simulink model "gtm_design"  (R2020b)
settings: Solver=ode3  StartTime=0.0  StopTime=20  FixedStep=Timestep  MaxStep=0.1  MinStep=0.005  RelTol=1e-5
StopFcn:
  | MWSout=grabmws(bdroot);
  | MWSout.lastrun=datestr(now);
values from neighbouring files (symbols this model uses):
  AILL = simout.surf.AILL.Data    [plot_result.m]
  AILR = simout.surf.AILR.Data    [plot_result.m]
  ELLIB = simout.surf.ELLIB.Data    [plot_result.m]
  ELLOB = simout.surf.ELLOB.Data    [plot_result.m]
  ELRIB = simout.surf.ELRIB.Data    [plot_result.m]
  ELROB = simout.surf.ELROB.Data    [plot_result.m]
  RUDL = simout.surf.RUDL.Data    [plot_result.m]
  RUDU = simout.surf.RUDU.Data    [plot_result.m]
  THROTL = simout.surf.THROTL.Data    [plot_result.m]
  THROTR = simout.surf.THROTR.Data    [plot_result.m]
undefined symbols (not defined in the file or in its folder): Aero, aftfuel, aftfuel_pos, AILLC, AILRC, alpha_deg, altitude_ft, Ax_g, Ay_g, Az_g, b, beta_deg, bias, BRAKEC, Cbar, cg_pos0, cg_shift_gear, DamageCase, DamageModels, DamageOnsetTime, ELLIBC, ELLOBC, ELRIBC, ELROBC, engl_ang, engl_pos, engr_ang, engr_pos, FLAPLIB, FLAPLIC, FLAPLOB, FLAPLOC, FLAPRIB, FLAPRIC, FLAPROB, FLAPROC, FuelUsed_Init, fwdfuel, fwdfuel_pos, GEAR, GEARC, Inertia0, Inertia_shift_gear, Ixx_model, Iyy_model, Izz_model, KTAS, LandingGear, LengON, LinearizeModeOn, NAV_altitude_m, NAV_latitude_deg, NAV_longitude_deg, NAV_Ve_mps, NAV_Vn_mps, NAV_Vu_mps, Newton, p_deg, phi_deg, POS_hi ... (+40)
libraries: simulink_need_slupdate x40, simulink x4, simulink_extras x3, UserContent_lib x1
(part 1 of 6)
settings Model: ExtModeAutoUpdateStatusClock=off  OrderedModelArguments=off  Creator=cox  LastModifiedBy=Jihoon Lee
settings DataIOCC: LimitDataPoints=on  MaxDataPoints=50000  SaveFormat=Structure  SaveOutput=off  DSMLogging=off  ReturnWorkspaceOutputs=off
settings OptimizationCC: BooleanDataType=off  ExpressionDepthLimit=2147483647  InitFltsAndDblsToZero=on  LifeSpan=inf
settings DebuggingCC: AlgebraicLoopMsg=error  SaveWithParameterizedLinksMsg=none  MergeDetectMultiDrivingBlocksExec=none  SignalResolutionControl=TryResolveAllWithWarning  InheritedTsInSrcMsg=none  MultiTaskDSMMsg=warning  MultiTaskCondExecSysMsg=none  StateNameClashWarn=warning  InitInArrayFormatMsg=none  SFUnexpectedBacktrackingDiag=warning  SFNoUnconditionalDefaultTransitionDiag=warning  SFExecutionAtInitializationDiag=none  ArithmeticOperatorsInVariantConditions=warning
settings HardwareCC: ProdBitPerPointer=32  ProdBitPerSizeT=32  ProdBitPerPtrDiffT=32  ProdLargestAtomicFloat=None  ProdIntDivRoundTo=Undefined  ProdEndianess=Unspecified  ProdWordSize=32  ProdHWDeviceType=32-bit Generic  TargetHWDeviceType=32-bit Generic
settings ModelReferenceCC: PropagateSignalLabelsOutOfModel=off
settings SFSimCC: SimUseLocalCustomCode=off  SimParseCustomCode=off  CustomCodeUndefinedFunction=UseInterfaceOnly
settings RTWCC: RTWUseLocalCustomCode=off
settings CodeAppCC: StateflowObjectComments=on
settings GRTTargetCC: TargetFcnLib=ansi_tfl_tmw.mat  TargetLangStandard=C89/C90 (ANSI)  CombineOutputUpdateFcns=off  GRTInterface=on
settings ConfigComp: CovMetricSettings=dw  CovSaveCumulativeToWorkspaceVar=on  CovSaveSingleToWorkspaceVar=on  CovExternalEMLEnable=off

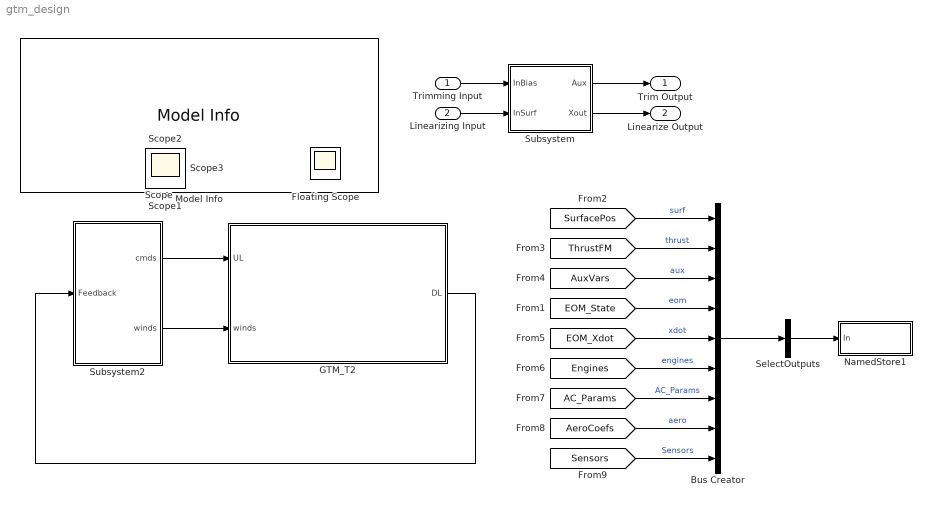
== system gtm_design ==
  Trimming Input : Inport  OutDataTypeStr=double  PortDimensions=4
  Linearizing Input : Inport  Port=2  OutDataTypeStr=double  PortDimensions=19
  Bus Creator : BusCreator  Inputs=9
  GTM_T2 : Subsystem  Tag=From trunk/GTMsim/gtm_model.mdl revision 162
      mask Display: image('GTMtiny.png')
  Model Info : simulink/Model-Wide Utilities/Model Info  Frame=on  DisplayStringWithTags=|  HorizontalTextAlignment=Center  LeftAlignmentValue=0.5
      | GTM Design-Simulation Model
      | Release 13-08
      | Last modified by %<LastModifiedBy> on %<LastModificationDate>
      | 
      | Copyright 2009
      | United States Government as represented by the 
      | Administrator of the National and Aeronautics and Space Administration.
      | 
      | No copyright is claimed in the United States under Title 17, U.S. Code.
      | All Other Rights Reserved.
  NamedStore1 : Subsystem  StopFcn=|  mask{enable_logging=on, do_stopfcn_callback=on}
      | if strmatch(get_param(gcb,'do_stopfcn_callback'),...
      | 'on','exact')                                       
      |    if exist('logsout','var')                        
      |        sout = CreateSimOut(logsout);                
      |    else                                             
      |         %disp('No Log Data Variable')               
      |     end                                             
      | clear logsout                                       
      | end
      mask prompts: enable_logging "Enable Data Logging"; do_stopfcn_callback "Post-process logsout"
      mask help: Produces signal log of input data. If post processing is selected the logsout object is converted into a data structure (sout) with fields named after the bus signals. In this case a common time base is recommended.
      mask init:
      | H=get_param([gcb,'/In'],'PortHandles');
      | if (enable_logging)
      |     set(H.Outport(1),'DataLogging','on')
      | else
      |     set(H.Outport(1),'DataLogging','off')
      |     
      | end
  SelectOutputs : BusSelector  OutputSignals=surf,thrust,aux,eom,xdot,engines,AC_Params,aero,Sensors  OutputAsBus=on
  Subsystem : Subsystem
  Subsystem2 : Subsystem
  Trim Output : Outport  OutDataTypeStr=double  PortDimensions=6  VectorParamsAs1DForOutWhenUnconnected=off
  Linearize Output : Outport  Port=2  OutDataTypeStr=double  PortDimensions=12  VectorParamsAs1DForOutWhenUnconnected=off
  Floating Scope : Scope
  Scope{,1..3} (4 alike) : Scope
  wires:
  SelectOutputs/1 -> NamedStore1/1(In)
  [SurfacePos] -> Bus Creator/1  "surf"
  Linearizing Input/1 -> Subsystem/2(InSurf)
  Subsystem/1(Aux) -> Trim Output/1
  [EOM_State] -> Bus Creator/4  "eom"
  [AuxVars] -> Bus Creator/3  "aux"
  [ThrustFM] -> Bus Creator/2  "thrust"
  Subsystem/2(Xout) -> Linearize Output/1
  [EOM_Xdot] -> Bus Creator/5  "xdot"
  [Engines] -> Bus Creator/6  "engines"
  [AC_Params] -> Bus Creator/7  "AC_Params"
  Bus Creator/1 -> SelectOutputs/1
  GTM_T2/1(DL) -> Subsystem2/1(Feedback)
  [AeroCoefs] -> Bus Creator/8  "aero"
  [Sensors] -> Bus Creator/9  "Sensors"
  Trimming Input/1 -> Subsystem/1(InBias)
  Subsystem2/1(cmds) -> GTM_T2/1(UL)
  Subsystem2/2(winds) -> GTM_T2/2(winds)

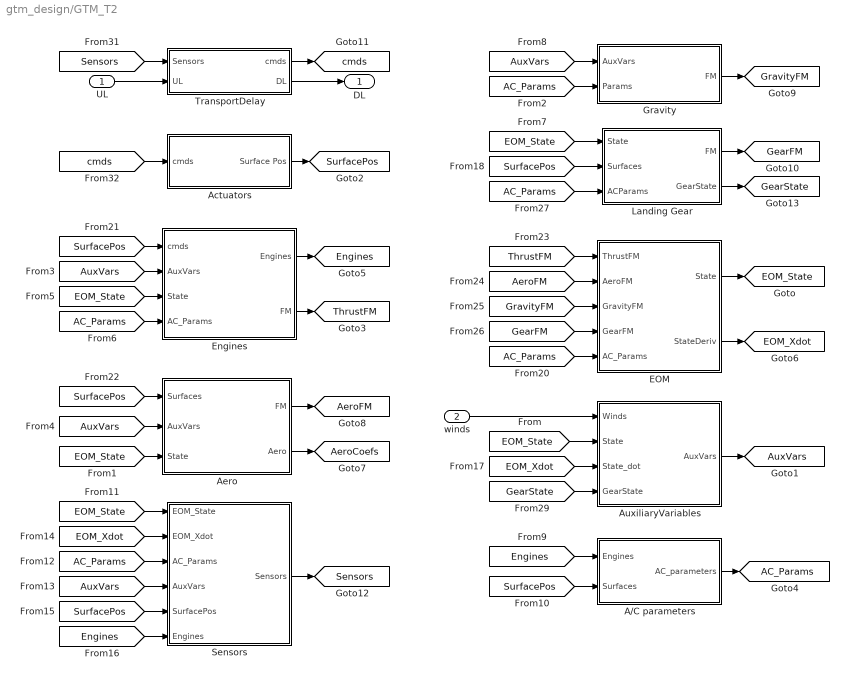
== system gtm_design/GTM_T2 ==
  UL : Inport
  winds : Inport  Port=2  PortDimensions=6
  A/C parameters : Subsystem
  Actuators : Subsystem
  Aero : Subsystem
  AuxiliaryVariables : Subsystem
  EOM : Subsystem
  Engines : Subsystem
  Gravity : Subsystem
  Landing Gear : Subsystem
  Sensors : Subsystem
  TransportDelay : Subsystem
  DL : Outport  VectorParamsAs1DForOutWhenUnconnected=off
  tag scope: AC_Params=global, AeroCoefs=global, AeroFM=global, AuxVars=global, EOM_State=global, EOM_Xdot=global, Engines=global, GearFM=global, GearState=global, GravityFM=global, Sensors=global, SurfacePos=global, ThrustFM=global, cmds=global
  wires:
  UL/1 -> TransportDelay/2(UL)
  TransportDelay/2(DL) -> DL/1
  Gravity/1(FM) -> [GravityFM]
  [AuxVars] -> Sensors/4(AuxVars)
  [EOM_Xdot] -> Sensors/2(EOM_Xdot)
  [Engines] -> Sensors/6(Engines)
  [SurfacePos] -> Sensors/5(SurfacePos)
  [AC_Params] -> Sensors/3(AC_Params)
  [EOM_State] -> Sensors/1(EOM_State)
  [AC_Params] -> EOM/5(AC_Params)
  [GearFM] -> EOM/4(GearFM)
  [GravityFM] -> EOM/3(GravityFM)
  [AeroFM] -> EOM/2(AeroFM)
  [ThrustFM] -> EOM/1(ThrustFM)
  [EOM_State] -> AuxiliaryVariables/2(State)
  Aero/2(Aero) -> [AeroCoefs]
  [SurfacePos] -> Aero/1(Surfaces)
  [AC_Params] -> Landing Gear/3(ACParams)
  [SurfacePos] -> Engines/1(cmds)
  EOM/2(StateDeriv) -> [EOM_Xdot]
  [EOM_Xdot] -> AuxiliaryVariables/3(State_dot)
  Engines/1(Engines) -> [Engines]
  [SurfacePos] -> A/C parameters/2(Surfaces)
  [Engines] -> A/C parameters/1(Engines)
  A/C parameters/1(AC_parameters) -> [AC_Params]
  [AC_Params] -> Engines/4(AC_Params)
  [AuxVars] -> Engines/2(AuxVars)
  [EOM_State] -> Engines/3(State)
  [AuxVars] -> Gravity/1(AuxVars)
  [AC_Params] -> Gravity/2(Params)
  EOM/1(State) -> [EOM_State]
  Engines/2(FM) -> [ThrustFM]
  Aero/1(FM) -> [AeroFM]
  [AuxVars] -> Aero/2(AuxVars)
  AuxiliaryVariables/1(AuxVars) -> [AuxVars]
  [EOM_State] -> Aero/3(State)
  [EOM_State] -> Landing Gear/1(State)
  [SurfacePos] -> Landing Gear/2(Surfaces)
  Landing Gear/1(FM) -> [GearFM]
  Actuators/1(Surface Pos) -> [SurfacePos]
  winds/1 -> AuxiliaryVariables/1(Winds)
  TransportDelay/1(cmds) -> [cmds]
  [Sensors] -> TransportDelay/1(Sensors)
  [cmds] -> Actuators/1(cmds)
  Sensors/1(Sensors) -> [Sensors]
  Landing Gear/2(GearState) -> [GearState]
  [GearState] -> AuxiliaryVariables/4(GearState)

== system gtm_design/NamedStore1 ==
  In : Inport
  To Workspace : ToWorkspace  VariableName=simout  SaveFormat=Timeseries  SampleTime=-1
  wires:
  In/1 -> To Workspace/1  "SimOut"

== system gtm_design/Subsystem ==
  InBias : Inport
  InSurf : Inport  Port=2
  Bus Selector : BusSelector  OutputSignals=eas,tas,alpha,beta,gamma,gndtrack  OutputAsBus=on
  Bus to Vector : BusToVector
  Bus to Vector1 : BusToVector
  DocBlock : simulink/Model-Wide Utilities/DocBlock  DocumentType=Text
      content=|
      | Inputs and Outputs selected here have a specific ordering.
      |
      |
      |
      | Do not change this without also changing output channel ordering in associated linmodel.m and
      | trimgtm.m functions
  Aux : Outport  VectorParamsAs1DForOutWhenUnconnected=off
  Xout : Outport  Port=2  VectorParamsAs1DForOutWhenUnconnected=off
  tag scope: SurfaceBias=global, SurfaceDeltas=global
  wires:
  [AuxVars] -> Bus Selector/1  "aux"
  [EOM_State] -> Bus to Vector1/1  "eom"
  Bus Selector/1 -> Bus to Vector/1
  InSurf/1 -> [SurfaceDeltas]
  Bus to Vector/1 -> Aux/1
  Bus to Vector1/1 -> Xout/1
  InBias/1 -> [SurfaceBias]

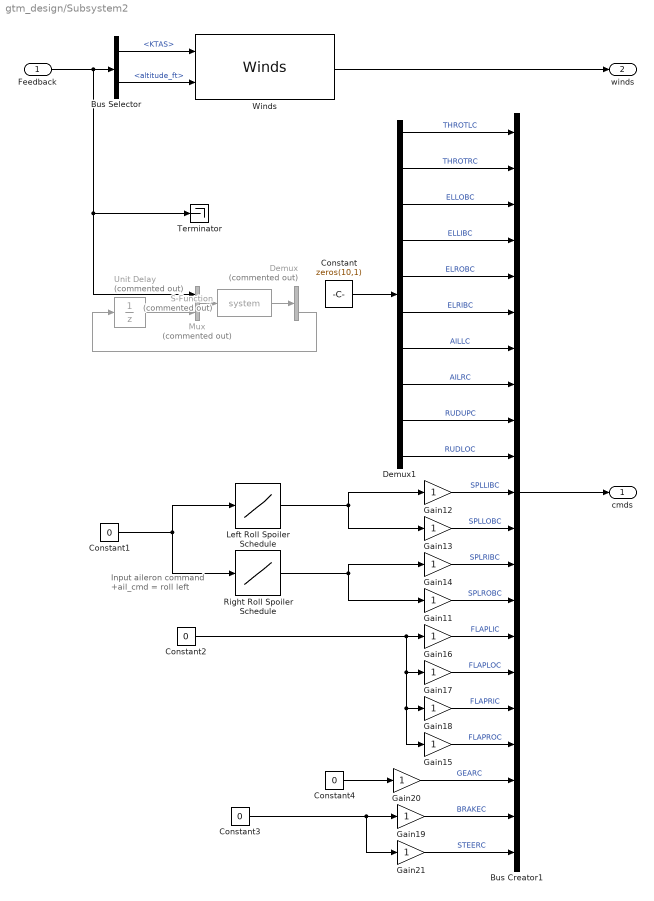
== system gtm_design/Subsystem2 ==
  note: Input aileron command
      | +ail_cmd = roll left
  Feedback : Inport
  Bus Creator1 : BusCreator  Inputs=21
  Bus Selector : BusSelector  OutputSignals=AirData.KTAS,AirData.altitude_ft
  Constant : Constant  Value=zeros(10,1)
  Constant{1..4} (4 alike) : Constant  Value=0
  Demux : Demux  Commented=on  Outputs=[10;9]
  Demux1 : Demux  Outputs=10
  Gain{11..21} (11 alike) : Gain  SaturateOnIntegerOverflow=on  OutDataTypeStr=Inherit: Same as input  ParamDataTypeStr=Inherit: Same as input
  Left Roll Spoiler Schedule : Lookup  InputValues="[-20\t-11.76\t-2.36\t0\t2.36\t11.76\t20\t]"  Table=[0 0 0 0 0 9 45]  LookUpMeth=Interpolation-Use End Values
  Mux : Mux  Commented=on  Inputs=[39;9]
  Right Roll Spoiler Schedule : Lookup  InputValues="[-20\t-11.76\t-2.36\t0\t2.36\t11.76\t20\t]"  Table=[45 9 0 0 0 0 0]  LookUpMeth=Interpolation-Use End Values
  S-Function : S-Function  Commented=on  SFunctionDeploymentMode=off  EnableBusSupport=off
  Terminator : Terminator
  Unit Delay : UnitDelay  Commented=on  SampleTime=-1  HasFrameUpgradeWarning=on
  Winds : UserContent_lib/Input Generator/Winds  WindSpeed_knots=WindSpd  WindDirection_deg=WindDir  level=None
  cmds : Outport
  winds : Outport  Port=2
  wires:
  Demux1/10 -> Bus Creator1/10  "RUDLOC"
  Gain19/1 -> Bus Creator1/20  "BRAKEC"
  Constant1/1 -> Left Roll Spoiler Schedule/1, Right Roll Spoiler Schedule/1
  Demux1/5 -> Bus Creator1/5  "ELROBC"
  Bus Selector/1 -> Winds/1  "<KTAS>"
  Gain12/1 -> Bus Creator1/11  "SPLLIBC"
  Feedback/1 -> Mux/1, Terminator/1, Bus Selector/1
  Gain16/1 -> Bus Creator1/15  "FLAPLIC"
  Demux1/3 -> Bus Creator1/3  "ELLOBC"
  Constant2/1 -> Gain15/1, Gain18/1, Gain17/1, Gain16/1
  Demux1/8 -> Bus Creator1/8  "AILRC"
  Gain21/1 -> Bus Creator1/21  "STEERC"
  Constant4/1 -> Gain20/1
  Constant3/1 -> Gain21/1, Gain19/1
  Demux1/1 -> Bus Creator1/1  "THROTLC"
  Right Roll Spoiler Schedule/1 -> Gain14/1, Gain11/1
  Demux1/2 -> Bus Creator1/2  "THROTRC"
  Demux1/9 -> Bus Creator1/9  "RUDUPC"
  Demux1/7 -> Bus Creator1/7  "AILLC"
  Gain20/1 -> Bus Creator1/19  "GEARC"
  Bus Selector/2 -> Winds/2  "<altitude_ft>"
  Demux1/4 -> Bus Creator1/4  "ELLIBC"
  Bus Creator1/1 -> cmds/1
  Gain17/1 -> Bus Creator1/16  "FLAPLOC"
  Winds/1 -> winds/1
  Gain11/1 -> Bus Creator1/14  "SPLROBC"
  Gain18/1 -> Bus Creator1/17  "FLAPRIC"
  Demux1/6 -> Bus Creator1/6  "ELRIBC"
  Left Roll Spoiler Schedule/1 -> Gain12/1, Gain13/1
  Gain13/1 -> Bus Creator1/12  "SPLLOBC"
  Gain15/1 -> Bus Creator1/18  "FLAPROC"
  Gain14/1 -> Bus Creator1/13  "SPLRIBC"
  Constant/1 -> Demux1/1
  Mux/1 -> S-Function/1
  Unit Delay/1 -> Mux/2
  Demux/2 -> Unit Delay/1
  S-Function/1 -> Demux/1

== system gtm_design/GTM_T2/A//C parameters ==
  Engines : Inport
  Surfaces : Inport  Port=2
  B : Constant  Value=b
  Bus Creator4 : BusCreator  Inputs=15
  Bus Selector : BusSelector  OutputSignals=fuel_used
  Cbar : Constant  Value=Cbar
  Demux : Demux  Outputs=6
  Inertia/Mass/CG Shift : Subsystem  mask{DamageModels=DamageModels}
      mask prompts: DamageModels "Array of Damage Cases"
      mask init:
      | Ncases=length(DamageModels);
      | dCGDamage=zeros(Ncases+1,3);   
      | dMassDamage=zeros(Ncases+1,1);
      | dInertiaDamage=zeros(Ncases+1,6);
      | for i=1:Ncases,
      |   if isfield(DamageModels{i},'Mass'),
      |      dInertiaDamage(i+1,:)=DamageModels{i}.Mass.dIxxIyyIzzIxzIyzIxy;
      |      dCGDamage(i+1,:)=DamageModels{i}.Mass.dCG;
      |      dMassDamage(i+1)=DamageModels{i}.Mass.dWeight;
      |   end
      | end
  S : Constant  Value=S
  TriggerDamage : Subsystem
  ixxb5 : Constant  Value=engr_pos
  ixxb6 : Constant  Value=engl_pos
  xCG1 : Constant  Value=ref_cg
  AC_parameters : Outport  VectorParamsAs1DForOutWhenUnconnected=off
  wires:
  Bus Selector/1 -> Inertia/Mass/CG Shift/2(fuel_used)  "<fuel_used>"
  [DamageCase] -> Inertia/Mass/CG Shift/3(DamageCase)
  [DamageCase] -> Bus Creator4/13  "DamageCase"
  Inertia/Mass/CG Shift/3(CG) -> Bus Creator4/12  "CG"
  Inertia/Mass/CG Shift/2(mass) -> Bus Creator4/11  "mass"
  Demux/6 -> Bus Creator4/10  "Ixy"
  Demux/5 -> Bus Creator4/9  "Iyz"
  Demux/4 -> Bus Creator4/8  "Ixz"
  Demux/3 -> Bus Creator4/7  "Izz"
  Demux/2 -> Bus Creator4/6  "Iyy"
  Demux/1 -> Bus Creator4/5  "Ixx"
  ixxb6/1 -> Bus Creator4/15  "LfEng"
  ixxb5/1 -> Bus Creator4/14  "RtEng"
  xCG1/1 -> Bus Creator4/4  "CP"
  B/1 -> Bus Creator4/3  "B"
  Cbar/1 -> Bus Creator4/2  "Cbar"
  S/1 -> Bus Creator4/1  "S"
  TriggerDamage/1(damagecase) -> [DamageCase]
  Inertia/Mass/CG Shift/1(Inertia) -> Demux/1
  Surfaces/1 -> Inertia/Mass/CG Shift/1(Surfaces)
  Engines/1 -> Bus Selector/1
  Bus Creator4/1 -> AC_parameters/1

== system gtm_design/GTM_T2/Actuators ==
  cmds : Inport
  Acutator Dynamics : Subsystem
  DeadBand : Subsystem
  InputModification for Trimming : Subsystem
  Label : Subsystem
  TimeDelay with IC feedthrough : Subsystem
  Surface Pos : Outport  VectorParamsAs1DForOutWhenUnconnected=off
  wires:
  TimeDelay with IC feedthrough/1(O) -> InputModification for Trimming/1(CmdVec)
  DeadBand/1(O) -> Surface Pos/1
  cmds/1 -> Acutator Dynamics/1(In)
  [SurfaceDeltas] -> InputModification for Trimming/3(SurfaceDeltas)
  Label/1(O) -> DeadBand/1(I)
  [SurfaceBias] -> InputModification for Trimming/2(SurfBias)
  InputModification for Trimming/1(CmdVecOut) -> Label/1(I)
  Acutator Dynamics/1(Out) -> TimeDelay with IC feedthrough/1(I)

== system gtm_design/GTM_T2/Aero ==
  Surfaces : Inport
  AuxVars : Inport  Port=2
  State : Inport  Port=3
  Basic Airframe : Subsystem
  Bus Selector1 : BusSelector  OutputSignals=CG,CP
  Bus Selector2 : BusSelector  OutputSignals=alpha,beta
  Bus Selector3 : BusSelector  OutputSignals=alpha  OutputAsBus=on
  Bus Selector4 : BusSelector  OutputSignals=beta  OutputAsBus=on
  Bus Selector6 : BusSelector  OutputSignals=tas
  Bus Selector7 : BusSelector  OutputSignals=qbar
  Bus Selector8 : BusSelector  OutputSignals=pb,qb,rb  OutputAsBus=on
  Bus to Vector5 : BusToVector
  Coefficent Evaluation : Subsystem  mask{b=b, cbar=Cbar, Sref=S}
      mask prompts: b "Reference Span (b)"; cbar "Reference Chord (cbar)"; Sref "Reference Area (Sref)"
      mask help:
      | Calulates the Force and Moments due to aerodynamic loads from vector of body axes aerodynamic coefficients:
      |    C6body = [Cx Cy Cz Cl Cm Cn].
      | Also requires dynamic pressure, cg/cp locations and reference lengths/area.
  Control Surfaces : Subsystem
  Dynamic Derviatives : Subsystem
  Label : Subsystem
  Stall Rolling Moment Asymmetry : Subsystem
  Sum8 : Sum  Inputs=++++  InputSameDT=on  SaturateOnIntegerOverflow=on  OutDataTypeStr=Inherit: Same as first input
  stall_cl_asym_enabled : Constant  Value=stall_cl_asym_enabled
  symmetry_on : Constant  Value=symmetric_aero_on
  FM : Outport  VectorParamsAs1DForOutWhenUnconnected=off
  Aero : Outport  Port=2  VectorParamsAs1DForOutWhenUnconnected=off
  wires:
  [AC_Params] -> Dynamic Derviatives/5(AC_Params)
  Bus to Vector5/1 -> Control Surfaces/5(pqr), Dynamic Derviatives/4(pqr)
  Bus Selector6/1 -> Control Surfaces/3(TAS), Dynamic Derviatives/3(TAS)  "<tas>"
  [AC_Params] -> Control Surfaces/6(AC_Params)
  [AC_Params] -> Basic Airframe/4(AC_Params)
  Bus Selector8/1 -> Bus to Vector5/1  "pqr"
  Basic Airframe/1(C6) -> Sum8/1
  Control Surfaces/1(dC6) -> Sum8/2
  Dynamic Derviatives/1(dC6) -> Sum8/3
  State/1 -> Bus Selector8/1
  Bus Selector2/2 -> Basic Airframe/2(beta), Dynamic Derviatives/2(beta), Control Surfaces/2(beta)  "<beta>"
  Bus Selector2/1 -> Basic Airframe/1(alpha), Dynamic Derviatives/1(alpha), Control Surfaces/1(alpha)  "<alpha>"
  AuxVars/1 -> Bus Selector2/1, Bus Selector6/1, Bus Selector3/1, Bus Selector7/1, Bus Selector4/1
  Label/1(O) -> FM/1
  Bus Selector7/1 -> Coefficent Evaluation/2(qbar)  "<qbar>"
  Sum8/1 -> Aero/1, Coefficent Evaluation/1(C6 Body)
  Coefficent Evaluation/1(Forces) -> Label/1(If)
  Coefficent Evaluation/2(Moments) -> Label/2(Im)
  Bus Selector1/1 -> Coefficent Evaluation/3(Cg)  "<CG>"
  [AC_Params] -> Bus Selector1/1
  Bus Selector1/2 -> Coefficent Evaluation/4(Cp)  "<CP>"
  symmetry_on/1 -> Basic Airframe/3(symmetry_on)
  Surfaces/1 -> Control Surfaces/4(surfaces)
  stall_cl_asym_enabled/1 -> Stall Rolling Moment Asymmetry/3(stall_cl_asym_enabled)
  Stall Rolling Moment Asymmetry/1(dC6) -> Sum8/4
  Bus Selector3/1 -> Stall Rolling Moment Asymmetry/1(alpha)
  Bus Selector4/1 -> Stall Rolling Moment Asymmetry/2(beta)

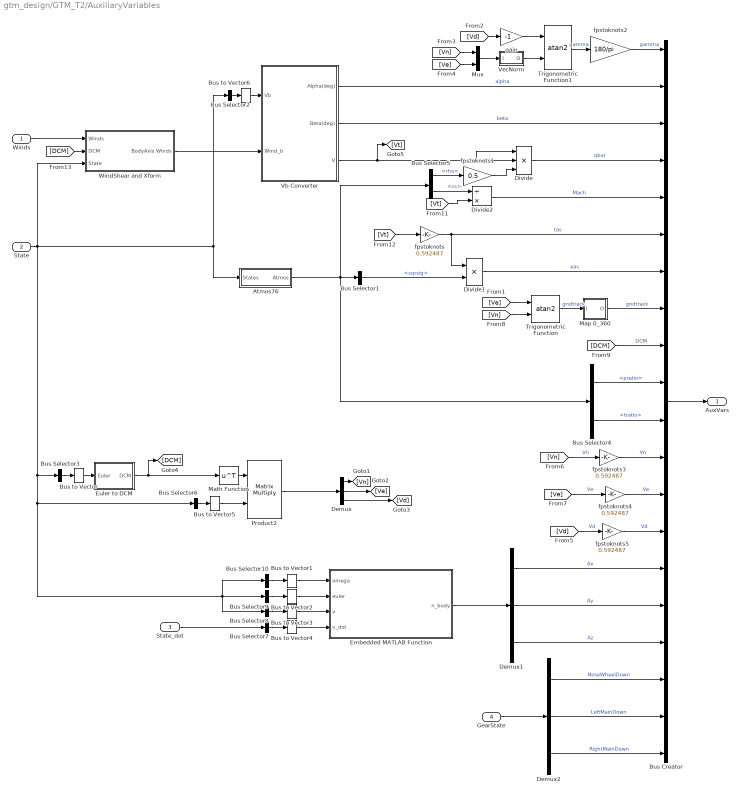
== system gtm_design/GTM_T2/AuxiliaryVariables ==
  Winds : Inport  PortDimensions=6
  State : Inport  Port=2
  State_dot : Inport  Port=3
  GearState : Inport  Port=4
  Atmos76 : Subsystem
  Bus Creator : BusCreator  Inputs=20
  Bus Selector1 : BusSelector  OutputSignals=sqrsig
  Bus Selector10 : BusSelector  OutputSignals=pb,qb,rb  OutputAsBus=on
  Bus Selector2 : BusSelector  OutputSignals=ub,vb,wb  OutputAsBus=on
  Bus Selector3 : BusSelector  OutputSignals=phi,theta,psi  OutputAsBus=on
  Bus Selector4 : BusSelector  OutputSignals=pratio,tratio
  Bus Selector5 : BusSelector  OutputSignals=rho,cs
  Bus Selector6 : BusSelector  OutputSignals=ub,vb,wb  OutputAsBus=on
  Bus Selector7 : BusSelector  OutputSignals=ub_dot,vb_dot,wb_dot  OutputAsBus=on
  Bus Selector8 : BusSelector  OutputSignals=ub,vb,wb  OutputAsBus=on
  Bus Selector9 : BusSelector  OutputSignals=phi,theta,psi  OutputAsBus=on
  Bus to Vector{,1..6} (7 alike) : BusToVector
  Demux : Demux  Outputs=3
  Demux1 : Demux  Outputs=3
  Demux2 : Demux  Outputs=3
  Divide : Product  Inputs=***
  Divide1 : Product
  Divide2 : Product  Inputs=/*
  Embedded MATLAB Function : MATLAB Function  TreatAsAtomicUnit=on
  Euler to DCM : Subsystem
  Map 0_360 : Subsystem
  Math Function : Math  Operator=transpose  SignedPower=on  SaturateOnIntegerOverflow=on
  Mux : Mux  Inputs=2
  Product2 : Product  Multiplication=Matrix(*)  RndMeth=Zero
  Trigonometric Function : Trigonometry  Operator=atan2
  Trigonometric Function1 : Trigonometry  Operator=atan2
  Vb Converter : Subsystem
  VecNorm : Subsystem
  WindShear and Xform : Subsystem
  fpstoknots{,3..5} (4 alike) : Gain  Gain=0.592487
  fpstoknots1 : Gain  Gain=0.5
  fpstoknots2 : Gain  Gain=180/pi
  gain : Gain  Gain=-1
  AuxVars : Outport  VectorParamsAs1DForOutWhenUnconnected=off
  wires:
  Demux2/3 -> Bus Creator/20  "RightMainDown"
  Demux2/2 -> Bus Creator/19  "LeftMainDown"
  Demux2/1 -> Bus Creator/18  "NoseWheelDown"
  GearState/1 -> Demux2/1
  [DCM] -> WindShear and Xform/2(DCM)
  WindShear and Xform/1(BodyAxis Winds) -> Vb Converter/2(Wind_b)
  Winds/1 -> WindShear and Xform/1(Winds)
  Product2/1 -> Demux/1
  Bus to Vector6/1 -> Vb Converter/1(Vb)
  Bus Selector2/1 -> Bus to Vector6/1
  Bus to Vector5/1 -> Product2/2
  Bus to Vector4/1 -> Embedded MATLAB Function/4(v_dot)
  Bus to Vector3/1 -> Embedded MATLAB Function/3(v)
  Bus to Vector2/1 -> Embedded MATLAB Function/2(euler)
  Bus to Vector1/1 -> Embedded MATLAB Function/1(omega)
  Bus to Vector/1 -> Euler to DCM/1("Euler ")
  Bus Selector3/1 -> Bus to Vector/1
  Bus Selector6/1 -> Bus to Vector5/1
  Math Function/1 -> Product2/1
  Demux/1 -> [Vn]
  Demux/2 -> [Ve]
  Embedded MATLAB Function/1(n_body) -> Demux1/1
  Demux1/3 -> Bus Creator/17  "Az"
  Demux1/2 -> Bus Creator/16  "Ay"
  Demux1/1 -> Bus Creator/15  "Ax"
  Bus Selector10/1 -> Bus to Vector1/1
  Bus Selector9/1 -> Bus to Vector2/1
  Bus Selector8/1 -> Bus to Vector3/1
  State_dot/1 -> Bus Selector7/1
  Bus Selector7/1 -> Bus to Vector4/1
  Bus Creator/1 -> AuxVars/1
  [Vt] -> fpstoknots/1
  [Vt] -> Divide2/2
  [DCM] -> Bus Creator/9  "DCM"
  fpstoknots5/1 -> Bus Creator/14  "Vd"
  fpstoknots4/1 -> Bus Creator/13  "Ve"
  fpstoknots3/1 -> Bus Creator/12  "Vn"
  Divide2/1 -> Bus Creator/5  "Mach"
  Bus Selector5/2 -> Divide2/1  "<cs>"
  Trigonometric Function/1 -> Map 0_360/1(I)  "gndtrack"
  Map 0_360/1(O) -> Bus Creator/8  "gndtrack"
  [Vn] -> Trigonometric Function/2
  [Ve] -> Trigonometric Function/1
  Bus Selector4/2 -> Bus Creator/11  "<tratio>"
  Bus Selector4/1 -> Bus Creator/10  "<pratio>"
  [Vd] -> fpstoknots5/1  "Vd"
  [Vn] -> fpstoknots3/1  "Vn"
  [Ve] -> fpstoknots4/1  "Ve"
  Divide1/1 -> Bus Creator/7  "eas"
  State/1 -> WindShear and Xform/3(State), Bus Selector3/1, Bus Selector6/1, Bus Selector8/1, Bus Selector10/1, Bus Selector9/1, Atmos76/1(States), Bus Selector2/1
  Atmos76/1(Atmos) -> Bus Selector4/1, Bus Selector1/1, Bus Selector5/1
  fpstoknots/1 -> Bus Creator/6, Divide1/1  "tas"
  Vb Converter/3(V) -> [Vt], Divide/1, Divide/2
  Bus Selector1/1 -> Divide1/2  "<sqrsig>"
  Vb Converter/1(Alpha(deg)) -> Bus Creator/2  "alpha"
  Vb Converter/2(Beta(deg)) -> Bus Creator/3  "beta"
  Bus Selector5/1 -> fpstoknots1/1  "<rho>"
  fpstoknots1/1 -> Divide/3
  Divide/1 -> Bus Creator/4  "qbar"
  Euler to DCM/1(DCM) -> Math Function/1, [DCM]
  Demux/3 -> [Vd]
  Trigonometric Function1/1 -> fpstoknots2/1  "gamma"
  gain/1 -> Trigonometric Function1/1
  [Vd] -> gain/1
  Mux/1 -> VecNorm/1(I)
  [Vn] -> Mux/1
  [Ve] -> Mux/2
  VecNorm/1(O) -> Trigonometric Function1/2
  fpstoknots2/1 -> Bus Creator/1  "gamma"

== system gtm_design/GTM_T2/EOM ==
  ThrustFM : Inport
  AeroFM : Inport  Port=2
  GravityFM : Inport  Port=3
  GearFM : Inport  Port=4
  AC_Params : Inport  Port=5
  Add : Sum  Inputs=++++
  Aircraft 6DOF : Subsystem  mask{UnitOfLength=ft}
      mask prompts: UnitOfLength "Length Unit"
      mask help:
      | Six Degree of Freedom Aircraft Simulation
      |
      | Input forces are both linear forces and torques -> [Fx Fy Fz Tl Tm Tn].
      | Inertia6 is a vector [Ixx Iyy Izz  Ixz Iyz Ixy], all positive
      | State Vector is [Vb pqr LatLonAlt PhiThetaPsi]
      mask init:
      | if (UnitOfLength==1), % ft
      |     Re=6.37043246e+06/.3048;
      | elseif (UnitOfLength==2), % m
      |     Re=6.37043246e+06;
      | end
      mask TypeOptions UnitOfLength: ft | meters
  Anti Windup : Subsystem
  Bus Selector1 : BusSelector  OutputSignals=Ixx,Iyy,Izz,Ixz,Iyz,Ixy  OutputAsBus=on
  Bus Selector11 : BusSelector  OutputSignals=mass
  Bus to Vector : BusToVector
  Bus to Vector1 : BusToVector
  Bus to Vector2 : BusToVector
  Integrator : Integrator  InitialCondition=StatesInp
  State Labels : Subsystem
  Xdot Labels : Subsystem
  State : Outport  VectorParamsAs1DForOutWhenUnconnected=off
  StateDeriv : Outport  Port=2  VectorParamsAs1DForOutWhenUnconnected=off
  wires:
  Bus to Vector2/1 -> Add/2
  Bus to Vector1/1 -> Add/1
  ThrustFM/1 -> Bus to Vector1/1
  AeroFM/1 -> Bus to Vector2/1
  State Labels/1(O) -> State/1
  Bus to Vector/1 -> Aircraft 6DOF/3(Inertia6)
  GearFM/1 -> Add/4
  GravityFM/1 -> Add/3
  Add/1 -> Aircraft 6DOF/1(Forces)
  Xdot Labels/1(O) -> StateDeriv/1
  Bus Selector1/1 -> Bus to Vector/1
  Aircraft 6DOF/1(Xdot) -> Xdot Labels/1(I), Integrator/1
  Anti Windup/1(O) -> State Labels/1(I)
  Integrator/1 -> Aircraft 6DOF/4(State), Anti Windup/1(I)
  Bus Selector11/1 -> Aircraft 6DOF/2(mass)  "<mass>"
  AC_Params/1 -> Bus Selector1/1, Bus Selector11/1

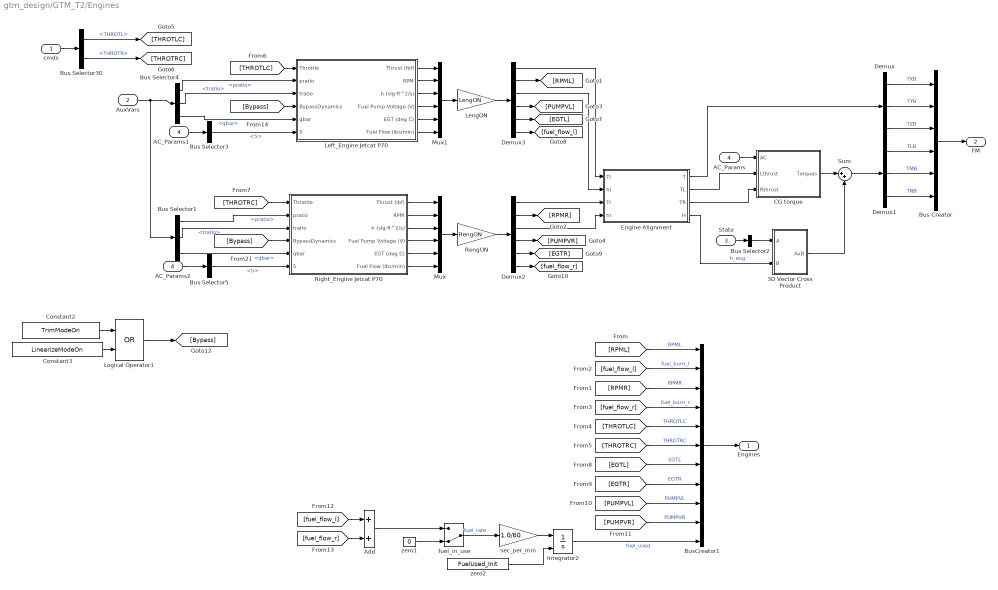
== system gtm_design/GTM_T2/Engines ==
  cmds : Inport
  AuxVars : Inport  Port=2
  State : Inport  Port=3
  AC_Params : Inport  Port=4
  3D Vector Cross Product : Subsystem
  AC_Params1 : InportShadow  Port=4
  AC_Params2 : InportShadow  Port=4
  Add : Sum
  Bus Creator : BusCreator  Inputs=6
  Bus Selector1 : BusSelector  OutputSignals=pratio,tratio,qbar
  Bus Selector2 : BusSelector  OutputSignals=pb,qb,rb  OutputAsBus=on
  Bus Selector3 : BusSelector  OutputSignals=S
  Bus Selector30 : BusSelector  OutputSignals=THROTL,THROTR
  Bus Selector4 : BusSelector  OutputSignals=pratio,tratio,qbar
  Bus Selector5 : BusSelector  OutputSignals=S
  BusCreator1 : BusCreator  Inputs=11
  CG torque : Subsystem
  Constant2 : Constant  Value=TrimModeOn
  Constant3 : Constant  Value=LinearizeModeOn
  Demux : Demux  Outputs=3
  Demux1 : Demux  Outputs=3
  Demux2 : Demux  Outputs=6
  Demux3 : Demux  Outputs=6
  Engine Alignment : MATLAB Function  TreatAsAtomicUnit=on
  Integrator2 : Integrator  InitialConditionSource=external
  Left_Engine Jetcat P70 : Subsystem
      mask init:
      | % Curve fit parameters for Jetcat P70 Model
      | % Coeff_thrust   = [0.000028864242464  -0.001914835880159 0.105916926095459  -1.251646340183624 ];
      | Coeff_thrust   = [0.000014847593013,  0, 0, 0.412662356277121];
      | Coeff_throttle = [0.000033035538475  -0.008354385314499 1.191126728328792 31.518959847101669];
      | Coeff_fuelflow = [0.000046800927870  -0.000779344124807 0.122178501497750];
      | Coeff_tau      = [ -2.2400e-02   2.9948e+00];
      | Coeff_EGT      = [ 2E-5, -0.0036,0.2342,-8.0496,664.99]; %EGT model, deg C
      | Coeff_dynamics = [ -.074 7.1];
      | fuelpump_table = [0 0.576	0.625	0.6985	0.7845	0.8575	0.919	0.9805	1.0415	1.1025...
      |                     1.1515	1.262	1.287	1.373	1.52	1.618	1.74	1.887	1.973...
      |                     2.12	2.255	2.4385	2.647	2.7575	2.9905	3.162]; %volts, table of fuel pump voltages
      | fuelflow_table = [0,0.0794,0.0876,0.102,0.1149,0.1275,0.1379,0.1487,0.1586,0.1671,...
      |                     0.1775,0.1858,0.194,0.2038,0.2206,0.2405,0.2566,0.2746,0.2921,0.3102,...
      |                     0.3266,0.3445,0.3533,0.3611,0.3866,0.4083;]*2; %lbs/min,   FULL fuel flow rates corresponding to pump voltages (fuelpump_table)  
      | % Equvalent Shaft parameters for engine
      | shaft_dia = 0.75/12.0;       % diameter of rotating turbine in feet 
      | shaft_len = 6.25/12.0;       % length of rotating turbine in feet   
      | density   = 15.2;            % mass density of steel in slugs/ft^3 
      | 
      | 
      | A = [-1.336,-0.7314;1,0;];
      | B = [1;0];
      | C = [-0.1474   0.7314];
      | D = 0;
  LengON : Gain  Gain=LengON  SaturateOnIntegerOverflow=on  OutDataTypeStr=Inherit: Same as input  ParamDataTypeStr=Inherit: Same as input
  Logical Operator1 : Logic  Operator=OR  AllPortsSameDT=off  OutDataTypeStr=boolean
  Mux : Mux  Inputs=6
  Mux1 : Mux  Inputs=6
  RengON : Gain  Gain=RengON  SaturateOnIntegerOverflow=on  OutDataTypeStr=Inherit: Same as input  ParamDataTypeStr=Inherit: Same as input
  Right_Engine Jetcat P70 : Subsystem
      mask init: same as gtm_design/GTM_T2/Engines/Left_Engine Jetcat P70
  Sum : Sum  Inputs=|++
  fuel_in_use : ManualSwitch  CurrentSetting=0
  sec_per_min : Gain  Gain=1.0/60.  SaturateOnIntegerOverflow=on  OutDataTypeStr=Inherit: Same as input  ParamDataTypeStr=Inherit: Same as input
  zero1 : Constant  Value=0
  zero2 : Constant  Value=FuelUsed_Init
  Engines : Outport  VectorParamsAs1DForOutWhenUnconnected=off
  FM : Outport  Port=2  PortDimensions=6  VectorParamsAs1DForOutWhenUnconnected=off
  wires:
  cmds/1 -> Bus Selector30/1
  Demux/2 -> Bus Creator/2  "TYB"
  State/1 -> Bus Selector2/1
  Bus Selector2/1 -> 3D Vector Cross Product/1(A)
  Demux/3 -> Bus Creator/3  "TZB"
  AuxVars/1 -> Bus Selector1/1, Bus Selector4/1
  AC_Params/1 -> CG torque/1(AC)
  Bus Creator/1 -> FM/1
  Bus Selector30/1 -> [THROTLC]  "<THROTL>"
  Bus Selector30/2 -> [THROTRC]  "<THROTR>"
  [THROTRC] -> BusCreator1/6  "THROTRC"
  [THROTLC] -> BusCreator1/5  "THROTLC"
  [fuel_flow_r] -> BusCreator1/4  "fuel_burn_r"
  [fuel_flow_l] -> BusCreator1/2  "fuel_burn_l"
  [RPMR] -> BusCreator1/3  "RPMR"
  [RPML] -> BusCreator1/1  "RPML"
  BusCreator1/1 -> Engines/1
  [EGTL] -> BusCreator1/7  "EGTL"
  [EGTR] -> BusCreator1/8  "EGTR"
  [PUMPVL] -> BusCreator1/9  "PUMPVL"
  [PUMPVR] -> BusCreator1/10  "PUMPVR"
  sec_per_min/1 -> Integrator2/1
  fuel_in_use/1 -> sec_per_min/1  "fuel_rate"
  Integrator2/1 -> BusCreator1/11  "fuel_used"
  zero2/1 -> Integrator2/2
  [fuel_flow_l] -> Add/1
  [fuel_flow_r] -> Add/2
  zero1/1 -> fuel_in_use/2
  Add/1 -> fuel_in_use/1
  Demux/1 -> Bus Creator/1  "TXB"
  Engine Alignment/4(H) -> 3D Vector Cross Product/2(B)  "h_eng"
  Engine Alignment/1(T) -> Demux/1
  Engine Alignment/2(TL) -> CG torque/2(Lthrust)
  Engine Alignment/3(TR) -> CG torque/3(Rthrust)
  CG torque/1(Torques) -> Sum/1
  3D Vector Cross Product/1(AxB) -> Sum/2
  Sum/1 -> Demux1/1
  Demux1/1 -> Bus Creator/4  "TLB"
  Demux1/2 -> Bus Creator/5  "TMB"
  Demux1/3 -> Bus Creator/6  "TNB"
  Mux/1 -> RengON/1
  RengON/1 -> Demux2/1
  Demux2/1 -> Engine Alignment/3(Tr)
  Demux2/2 -> [RPMR]
  Demux2/3 -> Engine Alignment/4(hr)
  Demux2/4 -> [PUMPVR]
  Demux2/5 -> [EGTR]
  Demux2/6 -> [fuel_flow_r]
  Mux1/1 -> LengON/1
  LengON/1 -> Demux3/1
  Demux3/1 -> Engine Alignment/1(Tl)
  Demux3/2 -> [RPML]
  Demux3/3 -> Engine Alignment/2(hl)
  Demux3/4 -> [PUMPVL]
  Demux3/5 -> [EGTL]
  Demux3/6 -> [fuel_flow_l]
  Constant3/1 -> Logical Operator1/2
  Constant2/1 -> Logical Operator1/1
  Logical Operator1/1 -> [Bypass]
  Left_Engine Jetcat P70/1(Thrust (lbf)) -> Mux1/1
  Left_Engine Jetcat P70/2(RPM) -> Mux1/2
  Left_Engine Jetcat P70/3(h (slg-ft^2/s)) -> Mux1/3
  Left_Engine Jetcat P70/4(Fuel Pump Voltage (V)) -> Mux1/4
  Left_Engine Jetcat P70/5(EGT (deg C)) -> Mux1/5
  Left_Engine Jetcat P70/6(Fuel Flow (lbs/min)) -> Mux1/6
  Right_Engine Jetcat P70/1(Thrust (lbf)) -> Mux/1
  Right_Engine Jetcat P70/2(RPM) -> Mux/2
  Right_Engine Jetcat P70/3(h (slg-ft^2/s)) -> Mux/3
  Right_Engine Jetcat P70/4(Fuel Pump Voltage (V)) -> Mux/4
  Right_Engine Jetcat P70/5(EGT (deg C)) -> Mux/5
  Right_Engine Jetcat P70/6(Fuel Flow (lbs/min)) -> Mux/6
  AC_Params2/1 -> Bus Selector5/1
  AC_Params1/1 -> Bus Selector3/1
  [THROTRC] -> Right_Engine Jetcat P70/1(Throttle)
  [THROTLC] -> Left_Engine Jetcat P70/1(Throttle)
  Bus Selector4/1 -> Left_Engine Jetcat P70/2(pratio)  "<pratio>"
  Bus Selector4/2 -> Left_Engine Jetcat P70/3(tratio)  "<tratio>"
  [Bypass] -> Left_Engine Jetcat P70/4(BypassDynamics)
  Bus Selector4/3 -> Left_Engine Jetcat P70/5(qbar)  "<qbar>"
  Bus Selector3/1 -> Left_Engine Jetcat P70/6(S)  "<S>"
  Bus Selector1/1 -> Right_Engine Jetcat P70/2(pratio)  "<pratio>"
  Bus Selector1/2 -> Right_Engine Jetcat P70/3(tratio)  "<tratio>"
  [Bypass] -> Right_Engine Jetcat P70/4(BypassDynamics)
  Bus Selector1/3 -> Right_Engine Jetcat P70/5(qbar)  "<qbar>"
  Bus Selector5/1 -> Right_Engine Jetcat P70/6(S)  "<S>"

== system gtm_design/GTM_T2/Gravity ==
  AuxVars : Inport
  Params : Inport  Port=2
  Bus Selector1 : BusSelector  OutputSignals=DCM
  Bus Selector6 : BusSelector  OutputSignals=mass
  Ground : Ground
  Ground1 : Ground
  Mux : Mux  Inputs=[3 3]
  Mux1 : Mux  Inputs=3
  Product : Product  Multiplication=Matrix(*)  RndMeth=Zero
  Product1 : Product  RndMeth=Zero
  acc due to gravity : Constant  Value=32.17405
  FM : Outport  VectorParamsAs1DForOutWhenUnconnected=off
  wires:
  acc due to gravity/1 -> Product1/2
  Ground1/1 -> Mux/2
  Product1/1 -> Mux1/3
  Ground/1 -> Mux1/2, Mux1/1
  Mux1/1 -> Product/2
  Mux/1 -> FM/1
  Product/1 -> Mux/1
  Params/1 -> Bus Selector6/1
  AuxVars/1 -> Bus Selector1/1
  Bus Selector1/1 -> Product/1  "<DCM>"
  Bus Selector6/1 -> Product1/1  "<mass>"

== system gtm_design/GTM_T2/Landing Gear ==
  State : Inport
  Surfaces : Inport  Port=2
  ACParams : Inport  Port=3
  Bus Selector : BusSelector  OutputSignals=BRAKE,STEER,GEAR
  Bus Selector1 : BusSelector  OutputSignals=pb,qb,rb  OutputAsBus=on
  Bus Selector2 : BusSelector  OutputSignals=ub,vb,wb  OutputAsBus=on
  Bus Selector3 : BusSelector  OutputSignals=psi
  Bus Selector4 : BusSelector  OutputSignals=altitude
  Bus Selector5 : BusSelector  OutputSignals=phi,theta,psi  OutputAsBus=on
  Bus Selector6 : BusSelector  OutputSignals=CG  OutputAsBus=on
  Bus to Vector : BusToVector
  Bus to Vector1 : BusToVector
  Bus to Vector2 : BusToVector
  Gain : Gain  Gain=1/100
  LandingGear : Subsystem  mask{NoseWheelPos=LandingGear.NoseWheelPos, LeftMainPos=LandingGear.LeftMainPos, RightMainPos=LandingGear.RightMainPos, SpringConst=LandingGear.SpringConst, DampingConst=LandingGear.DampingConst, StrokeLength=LandingGear.StrokeLength, MountStiffness=LandingGear.MountStiff, MountDamping=LandingGear.MountDamping, RunwayAlt=runway_alt}
      mask prompts: NoseWheelPos "Nose Wheel Position [X,Y,Z]"; LeftMainPos "Left Main Position [X,Y,Z]"; RightMainPos "Right Main Position [X,Y,Z]"; SpringConst "Spring Constant [Nose,Left,Right]"; DampingConst "Damping Constant [Nose,Left,Right]"; StrokeLength "Stroke Length [Nose,Left,Right]"; MountStiffness "Mount Stiffness [Nose,Left,Right]"; MountDamping "Mount Damping [Nose,Left, Right]"; RunwayAlt "Runway Altitude"
      mask help:
      | Implements ground reaction force (if geardown is nonzero) for 3-wheel landing gear. Linear stiffness and damping are applied within stroke range, and (generally larger) mount stiffness and damping are applied beyond this range.
      |
      | Underlying gear.c function is from HL-20/LaRCsim, e.b.jackson@nasa.gov
  Mux : Mux  Inputs=2
  FM : Outport  VectorParamsAs1DForOutWhenUnconnected=off
  GearState : Outport  Port=2  VectorParamsAs1DForOutWhenUnconnected=off
  wires:
  Mux/1 -> FM/1
  Gain/1 -> LandingGear/7(Brake (0-1))
  LandingGear/3(Contact) -> GearState/1
  LandingGear/2(M_gear) -> Mux/2
  LandingGear/1(F_gear) -> Mux/1
  Bus Selector/3 -> LandingGear/9(geardown (0/1))  "<GEAR>"
  Bus Selector/2 -> LandingGear/8(Steer (deg))  "<STEER>"
  Bus Selector/1 -> Gain/1  "<BRAKE>"
  Bus Selector3/1 -> LandingGear/6(Heading (Rad))  "<psi>"
  Bus to Vector/1 -> LandingGear/4(pqr (Rad/sec))
  Bus Selector4/1 -> LandingGear/3(Altitude (ft))  "<altitude>"
  Bus to Vector2/1 -> LandingGear/2(EulerAngles (Rad))
  Bus Selector6/1 -> LandingGear/1(cg)
  Surfaces/1 -> Bus Selector/1
  State/1 -> Bus Selector1/1, Bus Selector2/1, Bus Selector3/1, Bus Selector4/1, Bus Selector5/1
  Bus Selector1/1 -> Bus to Vector/1
  Bus to Vector1/1 -> LandingGear/5(Vbody (ft/sec))
  Bus Selector2/1 -> Bus to Vector1/1
  Bus Selector5/1 -> Bus to Vector2/1
  ACParams/1 -> Bus Selector6/1

== system gtm_design/GTM_T2/Sensors ==
  EOM_State : Inport
  EOM_Xdot : Inport  Port=2
  AC_Params : Inport  Port=3
  AuxVars : Inport  Port=4
  SurfacePos : Inport  Port=5
  Engines : Inport  Port=6
  Air Data : Subsystem
  AuxVars1 : InportShadow  Port=4
  Bus Creator : BusCreator  Inputs=5
  Engine ECU 8 Hz : Subsystem  SystemSampleTime=round(1/Timestep/8)*Timestep
  MAG3 IMU : Subsystem
  MIDG II 50 Hz : Subsystem  SystemSampleTime=round(1/Timestep/50)*Timestep
  Surface Pots : Subsystem
  Terminator : Terminator
  Terminator1 : Terminator
  Sensors : Outport  VectorParamsAs1DForOutWhenUnconnected=off
  wires:
  AC_Params/1 -> Terminator1/1
  EOM_Xdot/1 -> Terminator/1
  Bus Creator/1 -> Sensors/1
  Air Data/1(AirData) -> Bus Creator/1  "AirData"
  MIDG II 50 Hz/1(MIDG) -> Bus Creator/2  "MIDG"
  Surface Pots/1(Pots) -> Bus Creator/4  "SurfacePos"
  Engine ECU 8 Hz/1(ECU) -> Bus Creator/5  "Engines"
  MAG3 IMU/1(MAG3) -> Bus Creator/3  "MAG3"
  Engines/1 -> Engine ECU 8 Hz/1(Engines)
  SurfacePos/1 -> Surface Pots/1(SurfacePos)
  AuxVars/1 -> Air Data/2(AuxVars), MIDG II 50 Hz/1(AuxVars)
  EOM_State/1 -> MIDG II 50 Hz/2(EOM_State), Air Data/1(EOM_State), MAG3 IMU/2(EOM_State)
  AuxVars1/1 -> MAG3 IMU/1(AuxVars)

== system gtm_design/GTM_T2/TransportDelay ==
  note: Uplink Path
  note: Downlink Path
  Sensors : Inport
  UL : Inport  Port=2
  AntiAliasing : Subsystem
  Transport Delay on Bus : Subsystem
  Transport Delay on Bus1 : Subsystem
  cmds : Outport  VectorParamsAs1DForOutWhenUnconnected=off
  DL : Outport  Port=2  VectorParamsAs1DForOutWhenUnconnected=off
  wires:
  AntiAliasing/1(O) -> Transport Delay on Bus/1(In)
  Transport Delay on Bus/1(Out) -> DL/1
  UL/1 -> Transport Delay on Bus1/1(In)
  Sensors/1 -> AntiAliasing/1(I)
  Transport Delay on Bus1/1(Out) -> cmds/1

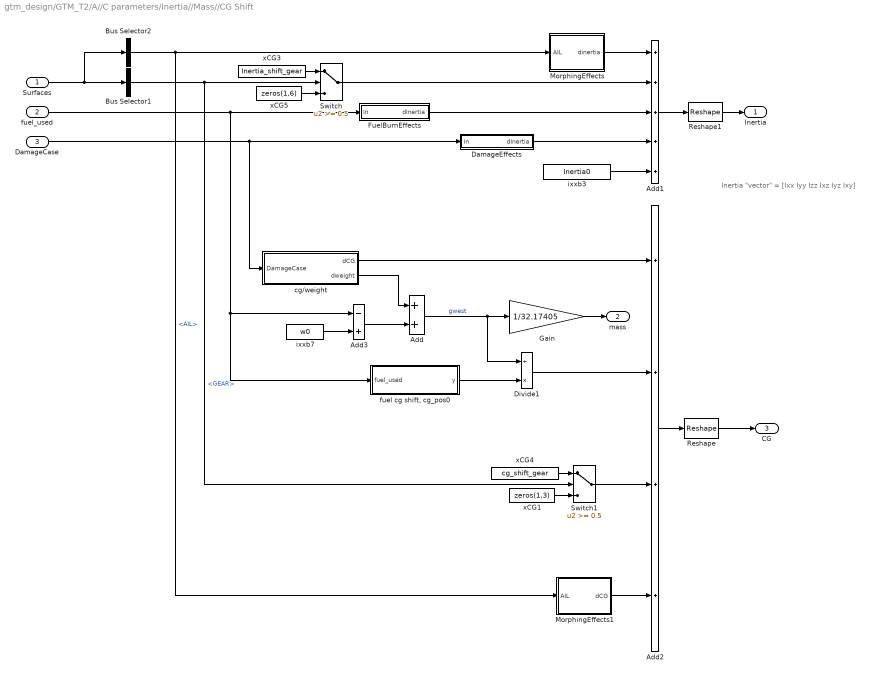
== system gtm_design/GTM_T2/A//C parameters/Inertia//Mass//CG Shift ==
  note: Inertia "vector" = [Ixx Iyy Izz Ixz Iyz Ixy]
  Surfaces : Inport
  fuel_used : Inport  Port=2
  DamageCase : Inport  Port=3
  Add : Sum
  Add1 : Sum  Inputs=+++++
  Add2 : Sum  Inputs=++++
  Add3 : Sum  Inputs=-+
  Bus Selector1 : BusSelector  OutputSignals=GEAR
  Bus Selector2 : BusSelector  OutputSignals=AILL,AILR  OutputAsBus=on
  DamageEffects : Subsystem
  Divide1 : Product  Inputs=/*
  FuelBurnEffects : Subsystem
  Gain : Gain  Gain=1/32.17405
  MorphingEffects : MATLAB Function  TreatAsAtomicUnit=on
  MorphingEffects1 : MATLAB Function  TreatAsAtomicUnit=on
  Reshape : Reshape
  Reshape1 : Reshape
  Switch : Switch  Threshold=0.5
  Switch1 : Switch  Threshold=0.5
  cg/weight : Subsystem
  "fuel cg shift, cg_pos0" : MATLAB Function  TreatAsAtomicUnit=on
  ixxb3 : Constant  Value=Inertia0
  ixxb7 : Constant  Value=w0
  xCG1 : Constant  Value=zeros(1,3)
  xCG3 : Constant  Value=Inertia_shift_gear
  xCG4 : Constant  Value=cg_shift_gear
  xCG5 : Constant  Value=zeros(1,6)
  Inertia : Outport  VectorParamsAs1DForOutWhenUnconnected=off
  mass : Outport  Port=2  VectorParamsAs1DForOutWhenUnconnected=off
  CG : Outport  Port=3  VectorParamsAs1DForOutWhenUnconnected=off
  wires:
  "fuel cg shift, cg_pos0"/1(y) -> Divide1/2
  Divide1/1 -> Add2/2
  Reshape1/1 -> Inertia/1
  Reshape/1 -> CG/1
  cg/weight/2(dweight) -> Add/1
  Bus Selector1/1 -> Switch1/2, Switch/2  "<GEAR>"
  cg/weight/1(dCG) -> Add2/1
  Add3/1 -> Add/2
  xCG1/1 -> Switch1/3
  xCG4/1 -> Switch1/1
  Switch1/1 -> Add2/3
  ixxb7/1 -> Add3/2
  Gain/1 -> mass/1
  Add2/1 -> Reshape/1
  Add/1 -> Divide1/1, Gain/1  "gwest"
  DamageCase/1 -> cg/weight/1(DamageCase), DamageEffects/1(In)
  DamageEffects/1(dInertia) -> Add1/4
  ixxb3/1 -> Add1/5
  fuel_used/1 -> "fuel cg shift, cg_pos0"/1(fuel_used), Add3/1, FuelBurnEffects/1(In)
  xCG5/1 -> Switch/3
  xCG3/1 -> Switch/1
  Add1/1 -> Reshape1/1
  Switch/1 -> Add1/2
  FuelBurnEffects/1(dInertia) -> Add1/3
  Surfaces/1 -> Bus Selector2/1, Bus Selector1/1
  Bus Selector2/1 -> MorphingEffects1/1(AIL), MorphingEffects/1(AIL)  "<AIL>"
  MorphingEffects/1(dinertia) -> Add1/1
  MorphingEffects1/1(dCG) -> Add2/4

== system gtm_design/GTM_T2/A//C parameters/TriggerDamage ==
  Clock : Clock
  DamgeCase : Constant  Value=DamageCase
  Switch : Switch  Threshold=DamageOnsetTime
  Zero : Constant  Value=0
  damagecase : Outport  VectorParamsAs1DForOutWhenUnconnected=off
  wires:
  Clock/1 -> Switch/2
  Switch/1 -> damagecase/1
  Zero/1 -> Switch/3
  DamgeCase/1 -> Switch/1
